simulink model "Powertrain_Comparison"  (R2024b)
settings: Solver=FixedStepDiscrete  StartTime=0.0  StopTime=3600  FixedStep=1  RelTol=1e-3
InitFcn:
  | try; sc=find_system(bdroot,'LookUnderMasks','all','FollowLinks','on','BlockType','Scope'); for k=1:numel(sc); c=get_param(sc{k},'ScopeConfiguration'); try; c.AxesScaling='Auto'; catch; end; try; nd=prod(c.LayoutDimensions); catch; nd=1; end; for d=1:nd; try; c.ActiveDisplay=d; catch; end; try; c.ShowLegend=true; catch; end; end; end; catch; end
(part 2 of 4)

== system Powertrain_Comparison/Electric powertrain/Battery DC converter ==
  note: Battery DC converter
  note: BIDIRECTIONAL DC CONVERTER | DC request to battery current
      | Reuses battery Voc and R. I = 2P / (Voc + sqrt(Voc^2 - 4RP)); avoids a terminal-voltage algebraic loop.
      | Bidirectional conversion and regenerative operation are route-model additions; conversion efficiency is assumed.
  note: INPUT SIGNALS
  note: PARAMETERS AND SIGNAL SELECTION
  note: CALCULATIONS AND CONTROL
  note: OUTPUTS AND MONITORING
  dispatch : Inport  PortDimensions=4
  fuel_cell_bus : Inport  Port=2  PortDimensions=3
  battery_state : Inport  Port=3  PortDimensions=12
  limits : Inport  Port=4  PortDimensions=2
  parameters : Inport  Port=5  PortDimensions=52
  Battery terminal power request W : Fcn  Expr=1000*((u(1)>=0)*u(1)/(((u(2))+(0.000001)+abs((u(2))-(0.000001)))/2)+(u(1)<0)*u(1)*u(2))
  Bus power within available current limits kW : Fcn  Expr=((((u(1))+(-u(3))+abs((u(1))-(-u(3))))/2)+(u(2))-abs((((u(1))+(-u(3))+abs((u(1))-(-u(3))))/2)-(u(2))))/2
  Ideal battery boost duty ratio : Fcn  Expr=((((1-u(1)/(((u(2))+(0.000001)+abs((u(2))-(0.000001)))/2))+(0)+abs((1-u(1)/(((u(2))+(0.000001)+abs((u(2))-(0.000001)))/2))-(0)))/2)+(0.95)-abs((((1-u(1)/(((u(2))+(0.000001)+abs((u(2))-(0.000001)))/2))+(0)+abs((1-u(1)/(((u(2))+(0.000001)+abs((u(2))-(0.000001)))/2))-(0)))/2)-(0.95)))/2
  Required battery bus power kW : Fcn  Expr=u(1)-u(2)
  Stable power-to-current request A : Fcn  Expr=2*u(1)/(((u(2)+sqrt(((u(2)^2-4*u(3)*u(1))+abs(u(2)^2-4*u(3)*u(1)))/2))+(0.000001)+abs((u(2)+sqrt(((u(2)^2-4*u(3)*u(1))+abs(u(2)^2-4*u(3)*u(1)))/2))-(0.000001)))/2)
  charge : Fcn  Expr=u(2)
  combine Converter request : Mux  Inputs=3
  combine Current command : Mux  Inputs=1
  dis : Fcn  Expr=u(1)
  eta_bconv : Fcn  Expr=u(27)
  fc : Fcn  Expr=u(1)
  inputs current_request : Mux  Inputs=3
  inputs duty : Mux  Inputs=2
  inputs limited : Mux  Inputs=3
  inputs request : Mux  Inputs=2
  inputs terminal : Mux  Inputs=2
  load : Fcn  Expr=u(4)
  r : Fcn  Expr=u(4)
  vbus : Fcn  Expr=u(25)
  voc : Fcn  Expr=u(3)
  Current command : Outport  PortDimensions=1
  Converter request : Outport  Port=2  PortDimensions=3
  wires:
  [r] -> inputs current_request/3
  [limits] -> charge/1
  [dispatch] -> load/1
  [fuel_cell_bus] -> fc/1
  [limited] -> combine Converter request/2
  [request] -> combine Converter request/1
  [parameters] -> eta_bconv/1
  [eta_bconv] -> inputs terminal/2
  [duty] -> combine Converter request/3
  [load] -> inputs request/1
  [request] -> inputs limited/1
  [limited] -> inputs terminal/1
  Bus power within available current limits kW/1 -> [limited]
  [voc] -> inputs duty/1
  limits/1 -> [limits]
  [vbus] -> inputs duty/2
  parameters/1 -> [parameters]
  dispatch/1 -> [dispatch]
  [fc] -> inputs request/2
  [terminal] -> inputs current_request/1
  [parameters] -> vbus/1
  [limits] -> dis/1
  battery_state/1 -> [battery_state]
  Battery terminal power request W/1 -> [terminal]
  [voc] -> inputs current_request/2
  inputs request/1 -> Required battery bus power kW/1
  r/1 -> [r]
  [current_request] -> combine Current command/1
  [battery_state] -> voc/1
  [dis] -> inputs limited/2
  [charge] -> inputs limited/3
  inputs terminal/1 -> Battery terminal power request W/1
  [battery_state] -> r/1
  fuel_cell_bus/1 -> [fuel_cell_bus]
  charge/1 -> [charge]
  combine Converter request/1 -> Converter request/1
  eta_bconv/1 -> [eta_bconv]
  load/1 -> [load]
  fc/1 -> [fc]
  Required battery bus power kW/1 -> [request]
  dis/1 -> [dis]
  vbus/1 -> [vbus]
  inputs current_request/1 -> Stable power-to-current request A/1
  combine Current command/1 -> Current command/1
  inputs limited/1 -> Bus power within available current limits kW/1
  inputs duty/1 -> Ideal battery boost duty ratio/1
  voc/1 -> [voc]
  Stable power-to-current request A/1 -> [current_request]
  Ideal battery boost duty ratio/1 -> [duty]

== system Powertrain_Comparison/Electric powertrain/Battery power limits ==
  note: Battery power limits
  note: BATTERY POWER LIMITS | state-dependent safe power at the DC bus
      | Pdis = (Voc - R Idis) Idis. Pcharge = (Voc + R Ich) Ich. The converter applies its directional efficiency.
  note: INPUT SIGNALS
  note: PARAMETERS AND SIGNAL SELECTION
  note: CALCULATIONS AND CONTROL
  note: OUTPUTS AND MONITORING
  demand : Inport  PortDimensions=12
  parameters : Inport  Port=2  PortDimensions=52
  Available bus charge sink kW : Fcn  Expr=(((u(1)+u(2)*u(3))*u(3)/(1000*(((u(4))+(0.000001)+abs((u(4))-(0.000001)))/2)))+abs((u(1)+u(2)*u(3))*u(3)/(1000*(((u(4))+(0.000001)+abs((u(4))-(0.000001)))/2))))/2
  Available bus discharge kW : Fcn  Expr=(((u(1)-u(2)*u(3))*u(3)*u(4)/1000)+abs((u(1)-u(2)*u(3))*u(3)*u(4)/1000))/2
  Current before maximum-power point A : Fcn  Expr=((u(1))+(u(2)/(2*(((u(3))+(0.000001)+abs((u(3))-(0.000001)))/2)))-abs((u(1))-(u(2)/(2*(((u(3))+(0.000001)+abs((u(3))-(0.000001)))/2)))))/2
  combine Power limits : Mux  Inputs=2
  eta_bconv : Fcn  Expr=u(27)
  ich : Fcn  Expr=u(6)
  idis : Fcn  Expr=u(5)
  inputs ch_bus : Mux
  inputs dis_bus : Mux
  inputs idis_safe : Mux  Inputs=3
  r : Fcn  Expr=u(4)
  voc : Fcn  Expr=u(3)
  Power limits : Outport  PortDimensions=2
  wires:
  [idis] -> inputs idis_safe/1
  [demand] -> voc/1
  [voc] -> inputs ch_bus/1
  inputs ch_bus/1 -> Available bus charge sink kW/1
  [voc] -> inputs dis_bus/1
  [ich] -> inputs ch_bus/3
  [ch_bus] -> combine Power limits/2
  idis/1 -> [idis]
  [r] -> inputs dis_bus/2
  [dis_bus] -> combine Power limits/1
  inputs dis_bus/1 -> Available bus discharge kW/1
  [demand] -> idis/1
  [parameters] -> eta_bconv/1
  [idis_safe] -> inputs dis_bus/3
  [demand] -> r/1
  demand/1 -> [demand]
  inputs idis_safe/1 -> Current before maximum-power point A/1
  [eta_bconv] -> inputs dis_bus/4
  [r] -> inputs ch_bus/2
  r/1 -> [r]
  [voc] -> inputs idis_safe/2
  [eta_bconv] -> inputs ch_bus/4
  eta_bconv/1 -> [eta_bconv]
  parameters/1 -> [parameters]
  [demand] -> ich/1
  [r] -> inputs idis_safe/3
  voc/1 -> [voc]
  combine Power limits/1 -> Power limits/1
  ich/1 -> [ich]
  Available bus charge sink kW/1 -> [ch_bus]
  Current before maximum-power point A/1 -> [idis_safe]
  Available bus discharge kW/1 -> [dis_bus]

== system Powertrain_Comparison/Electric powertrain/Battery storage ==
  note: Battery storage
  note: BATTERY STORAGE | reused battery-management model
      | Open Battery management to edit its pack mask. Current positive = discharge, negative = charge.
      | State output contains delayed SOC/temperature and state-derived limits; actual output contains delivered current, voltage and
      | power.
  note: INPUT SIGNALS
  note: CALCULATIONS AND CONTROL
  note: OUTPUTS AND MONITORING
  current_request : Inport  PortDimensions=1
  ambient : Inport  Port=2  PortDimensions=1
  Battery management : Subsystem  Description=Copied and adapted native battery energy-management subsystem. 96s41p; nominal59.51232kWh. SOC, OCV, current restrictions, I2R losses, thermal state, terminal energy and exact OCV-based stored energy. All data remain illustrative. No external file dependencies.  mask(Battery management parameters){initial_soc_pct=90, initial_temp_C=25, ns=96, np=41, cell_capacity_Ah=4.2, cell_nominal_V=3.6, cell_resistance_ohm=0.016, cell_voltage_limits_V=[2.5 4.2], current_ratings_C=[2 2], soc_levels_pct=[15 20 80 95], charge_temp_limits_C=[0 10 35 45], discharge_temp_limits_C=[-20 0 45 55], mass_kg=341.6666666667, cp_J_kgK=900, conductance_W_K=35, coulombic_efficiencies=[1 1], ocv_soc_pct=[0 5 10 20 30 40 50 60 70 80 90 95 100], ocv_cell_V=[2.5 3.1 3.3 3.45 3.53 3.6 3.67 3.73 3.8 3.9 4.04 4.12 4.2]}
      mask prompts: initial_soc_pct "Initial state of charge (%)"; initial_temp_C "Initial battery temperature (degC)"; ns "Series-connected cell groups, Ns"; np "Parallel cells per group, Np"; cell_capacity_Ah "Capacity of ONE cell (Ah)"; cell_nominal_V "Nominal voltage of ONE cell (V)"; cell_resistance_ohm "Resistance of ONE cell (ohm)"; cell_voltage_limits_V "Cell voltage limits [minimum maximum] (V)"; current_ratings_C "Current ratings [charge discharge] (C-rate)"; soc_levels_pct "SOC levels [minimum reserve taper maximum] (%)"; charge_temp_limits_C "Charge temperatures [stop-low full-low full-high stop-high] (degC)"; discharge_temp_limits_C "Discharge temperatures [stop-low full-low full-high stop-high] (degC)"; mass_kg "Effective pack thermal mass (kg)"; cp_J_kgK "Effective specific heat (J/(kg.K))"; conductance_W_K "Heat transfer to ambient (W/K)"; coulombic_efficiencies "Coulombic efficiencies [charge discharge] (0 to 1)"; ocv_soc_pct "OCV lookup: SOC breakpoints (%)"; ocv_cell_V "OCV lookup: matching single-cell voltages (V)"
      mask help: Reused battery-management model. Positive current discharges; negative current charges. Defaults use a96s41p,59.51232kWh nominal pack. OCV, resistance, thermal data and operating limits are illustrative. Keep13 OCV points. Fixed sample time1s. Stop simulation before changing data.
      mask init:
      | % Embedded parameter definitions. This code is stored in the SLX, not an external file.
      | assert(isscalar(ns) && isfinite(ns) && ns>=1 && ns==fix(ns), 'Series groups must be a positive integer.');
      | assert(isscalar(np) && isfinite(np) && np>=1 && np==fix(np), 'Parallel cells must be a positive integer.');
      | assert(isscalar(cell_capacity_Ah) && isfinite(cell_capacity_Ah) && cell_capacity_Ah>0, 'Cell capacity must be positive.');
      | assert(isscalar(cell_nominal_V) && isfinite(cell_nominal_V) && cell_nominal_V>0, 'Nominal cell voltage must be positive.');
      | assert(isscalar(cell_resistance_ohm) && isfinite(cell_resistance_ohm) && cell_resistance_ohm>0, 'Cell resistance must be greater than zero.');
      | assert(numel(cell_voltage_limits_V)==2 && all(isfinite(cell_voltage_limits_V)) && cell_voltage_limits_V(1)>0 && cell_voltage_limits_V(2)>cell_voltage_limits_V(1), 'Enter increasing positive cell voltage limits [min max].');
      | assert(cell_nominal_V>=cell_voltage_limits_V(1) && cell_nominal_V<=cell_voltage_limits_V(2), 'Nominal voltage must lie within the cell voltage limits.');
      | assert(numel(current_ratings_C)==2 && all(isfinite(current_ratings_C)) && all(current_ratings_C>=0), 'Enter two nonnegative C-rates [charge discharge].');
      | assert(numel(soc_levels_pct)==4 && all(isfinite(soc_levels_pct)) && all(diff(soc_levels_pct)>0) && soc_levels_pct(1)>=0 && soc_levels_pct(4)<=100, 'SOC levels must increase: minimum < reserve < taper < maximum, within 0 to 100.');
      | assert(isscalar(initial_soc_pct) && isfinite(initial_soc_pct) && initial_soc_pct>=soc_levels_pct(1) && initial_soc_pct<=soc_levels_pct(4), 'Initial SOC must lie inside the operating SOC window.');
      | assert(isscalar(initial_temp_C) && isfinite(initial_temp_C), 'Initial temperature must be a finite scalar.');
      | assert(numel(charge_temp_limits_C)==4 && all(isfinite(charge_temp_limits_C)) && all(diff(charge_temp_limits_C)>0), 'Enter four increasing charge-temperature limits.');
      | assert(numel(discharge_temp_limits_C)==4 && all(isfinite(discharge_temp_limits_C)) && all(diff(discharge_temp_limits_C)>0), 'Enter four increasing discharge-temperature limits.');
      | assert(isscalar(mass_kg) && isfinite(mass_kg) && mass_kg>0 && isscalar(cp_J_kgK) && isfinite(cp_J_kgK) && cp_J_kgK>0, 'Mass and specific heat must be positive.');
      | assert(isscalar(conductance_W_K) && isfinite(conductance_W_K) && conductance_W_K>=0, 'Ambient conductance must not be negative.');
      | assert(numel(coulombic_efficiencies)==2 && all(isfinite(coulombic_efficiencies)) && all(coulombic_efficiencies>0) && all(coulombic_efficiencies<=1), 'Coulombic efficiencies must be in (0,1].');
      | assert(isvector(ocv_soc_pct) && isvector(ocv_cell_V) && numel(ocv_soc_pct)>=2 && numel(ocv_soc_pct)==numel(ocv_cell_V), 'OCV arrays must be equal-length vectors.');
      | assert(all(isfinite(ocv_soc_pct)) && all(isfinite(ocv_cell_V)) && all(diff(ocv_soc_pct)>0) && ocv_soc_pct(1)==0 && ocv_soc_pct(end)==100, 'OCV SOC breakpoints must increase from 0 to 100.');
      | assert(all(diff(ocv_cell_V)>=0) && all(ocv_cell_V>=cell_voltage_limits_V(1)) && all(ocv_cell_V<=cell_voltage_limits_V(2)), 'OCV voltages must be nondecreasing and within the cell voltage limits.');
      | initial_soc=initial_soc_pct/100;
      | soc_min=soc_levels_pct(1)/100; soc_reserve=soc_levels_pct(2)/100;
      | soc_taper=soc_levels_pct(3)/100; soc_max=soc_levels_pct(4)/100;
      | cell_min_V=cell_voltage_limits_V(1); cell_max_V=cell_voltage_limits_V(2);
      | charge_rate_C=current_ratings_C(1); discharge_rate_C=current_ratings_C(2);
      | charge_T1_C=charge_temp_limits_C(1); charge_T2_C=charge_temp_limits_C(2);
      | charge_T3_C=charge_temp_limits_C(3); charge_T4_C=charge_temp_limits_C(4);
      | discharge_T1_C=discharge_temp_limits_C(1); discharge_T2_C=discharge_temp_limits_C(2);
      | discharge_T3_C=discharge_temp_limits_C(3); discharge_T4_C=discharge_temp_limits_C(4);
      | eta_charge=coulombic_efficiencies(1); eta_discharge=coulombic_efficiencies(2);
      | ocv_soc=ocv_soc_pct/100;
      | dt_s=1;
      | 
      | % Added exact OCV-integral energy accounting for the comparison.
      | assert(numel(ocv_soc)==13, 'This version requires13 OCV breakpoints and13 voltages.');
      | ocv_soc = reshape(ocv_soc,1,[]);
      | ocv_cell_V = reshape(ocv_cell_V,1,[]);
      | energy_s = [ocv_soc(ocv_soc<initial_soc) initial_soc];
      | energy_v = interp1(ocv_soc,ocv_cell_V,energy_s,'linear');
      | initial_stored_energy_kWh = ns*np*cell_capacity_Ah*trapz(energy_s,energy_v)/1000;
      mask Display: disp('BATTERY MANAGEMENT\n\nSOC and temperature\nVoltage and current limits\nLosses and energy\n\nDouble-click: parameters')
  combine Battery actual : Mux  Inputs=7
  combine Battery state : Mux  Inputs=12
  Battery state : Outport  PortDimensions=12
  Battery actual : Outport  Port=2  PortDimensions=7
  wires:
  current_request/1 -> [current_request]
  ambient/1 -> [ambient]
  [b8] -> combine Battery actual/2
  [b10] -> combine Battery actual/4
  [b6] -> combine Battery state/6
  [ambient] -> Battery management/2(AMBIENT_C)
  [b12] -> combine Battery actual/6
  [current_request] -> Battery management/1(CURRENT_A)
  [b11] -> combine Battery actual/5
  [b9] -> combine Battery actual/3
  [b1] -> combine Battery state/1
  [b7] -> combine Battery actual/1
  [b19] -> combine Battery actual/7
  [b2] -> combine Battery state/2
  [b3] -> combine Battery state/3
  [b4] -> combine Battery state/4
  [b5] -> combine Battery state/5
  [b13] -> combine Battery state/7
  [b14] -> combine Battery state/8
  [b15] -> combine Battery state/9
  [b16] -> combine Battery state/10
  [b17] -> combine Battery state/11
  [b18] -> combine Battery state/12
  Battery management/17(Stored_energy_kWh) -> [b17]
  Battery management/1(SOC_fraction) -> [b1]
  Battery management/18(Initial_stored_energy_kWh) -> [b18]
  Battery management/2(Battery_temperature_C) -> [b2]
  Battery management/19(Ohmic_loss_energy_kWh) -> [b19]
  Battery management/3(Open_circuit_voltage_V) -> [b3]
  Battery management/4(Equivalent_resistance_ohm) -> [b4]
  Battery management/5(Discharge_limit_A) -> [b5]
  Battery management/6(Charge_limit_A) -> [b6]
  Battery management/7(Terminal_voltage_V) -> [b7]
  Battery management/8(Actual_current_A) -> [b8]
  Battery management/9(Terminal_power_W) -> [b9]
  Battery management/10(Discharged_energy_kWh) -> [b10]
  Battery management/11(Charged_energy_kWh) -> [b11]
  Battery management/12(Ohmic_heat_W) -> [b12]
  Battery management/13(Initial_SOC_fraction) -> [b13]
  Battery management/14(Nominal_energy_kWh) -> [b14]
  Battery management/15(Capacity_Ah) -> [b15]
  Battery management/16(Stored_energy_depletion_kWh) -> [b16]
  combine Battery actual/1 -> Battery actual/1
  combine Battery state/1 -> Battery state/1

== system Powertrain_Comparison/Electric powertrain/DC boost converter ==
  note: DC boost converter
  note: DC BOOST CONVERTER | fuel-cell module to regulated DC link
      | Reuses boost steady-state Vout = Vin / (1-D). Dynamic switching and fixed resistive bench load are replaced by bus demand.
  note: INPUT SIGNALS
  note: PARAMETERS AND SIGNAL SELECTION
  note: CALCULATIONS AND CONTROL
  note: OUTPUTS AND MONITORING
  demand : Inport  PortDimensions=3
  parameters : Inport  Port=2  PortDimensions=52
  Boost converter loss kW : Fcn  Expr=u(1)-u(2)
  Fuel cell delivered DC bus kW : Fcn  Expr=u(1)*u(2)
  Ideal boost duty ratio : Fcn  Expr=((((1-u(1)/(((u(2))+(0.000001)+abs((u(2))-(0.000001)))/2))+(0)+abs((1-u(1)/(((u(2))+(0.000001)+abs((u(2))-(0.000001)))/2))-(0)))/2)+(0.95)-abs((((1-u(1)/(((u(2))+(0.000001)+abs((u(2))-(0.000001)))/2))+(0)+abs((1-u(1)/(((u(2))+(0.000001)+abs((u(2))-(0.000001)))/2))-(0)))/2)-(0.95)))/2
  combine Converter signals : Mux  Inputs=3
  eta_fcconv : Fcn  Expr=u(30)
  fc_voltage : Fcn  Expr=u(52)
  inputs bus : Mux  Inputs=2
  inputs duty : Mux  Inputs=2
  inputs loss : Mux  Inputs=2
  module : Fcn  Expr=u(1)
  vbus : Fcn  Expr=u(25)
  Converter signals : Outport  PortDimensions=3
  wires:
  [module] -> inputs bus/1
  [parameters] -> eta_fcconv/1
  [parameters] -> vbus/1
  [duty] -> combine Converter signals/3
  [bus] -> combine Converter signals/1
  Ideal boost duty ratio/1 -> [duty]
  [demand] -> module/1
  eta_fcconv/1 -> [eta_fcconv]
  [loss] -> combine Converter signals/2
  parameters/1 -> [parameters]
  [eta_fcconv] -> inputs bus/2
  [module] -> inputs loss/1
  [bus] -> inputs loss/2
  combine Converter signals/1 -> Converter signals/1
  [fc_voltage] -> inputs duty/1
  [vbus] -> inputs duty/2
  inputs duty/1 -> Ideal boost duty ratio/1
  demand/1 -> [demand]
  [parameters] -> fc_voltage/1
  Boost converter loss kW/1 -> [loss]
  module/1 -> [module]
  vbus/1 -> [vbus]
  inputs bus/1 -> Fuel cell delivered DC bus kW/1
  inputs loss/1 -> Boost converter loss kW/1
  fc_voltage/1 -> [fc_voltage]
  Fuel cell delivered DC bus kW/1 -> [bus]

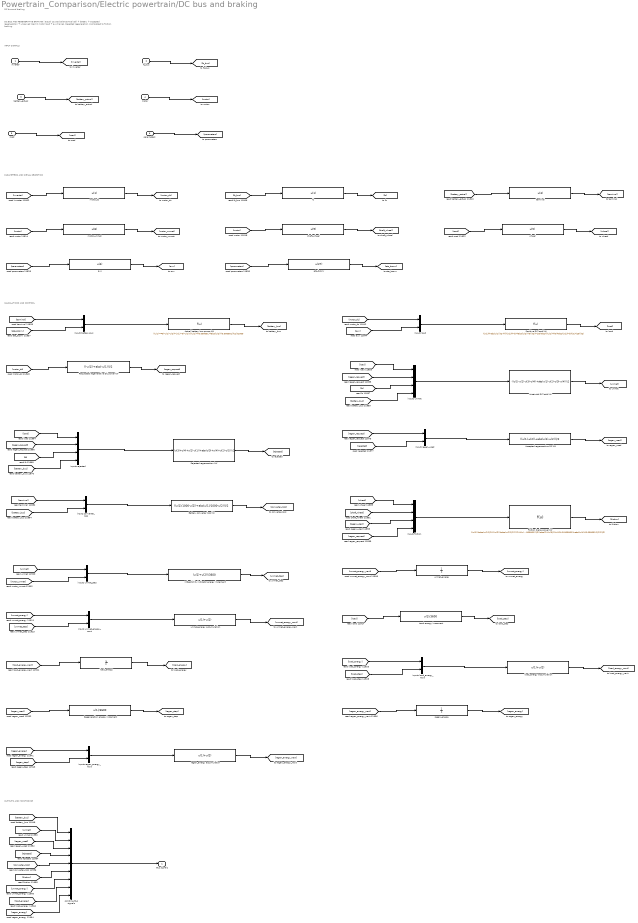
== system Powertrain_Comparison/Electric powertrain/DC bus and braking ==
  note: DC bus and braking
  note: DC BUS AND REGENERATIVE BRAKING | actual source balance
      | Fuel cell + battery + accepted regeneration + unserved load = motor load + auxiliaries. Rejected regeneration is allocated to
      | friction braking.
  note: INPUT SIGNALS
  note: PARAMETERS AND SIGNAL SELECTION
  note: CALCULATIONS AND CONTROL
  note: OUTPUTS AND MONITORING
  inverter : Inport  PortDimensions=2
  fc_bus : Inport  Port=2  PortDimensions=3
  battery_actual : Inport  Port=3  PortDimensions=7
  motor : Inport  Port=4  PortDimensions=9
  road : Inport  Port=5  PortDimensions=9
  parameters : Inport  Port=6  PortDimensions=52
  Accepted regenerative DC kW : Fcn  Expr=((u(1)-u(2))+abs(u(1)-u(2)))/2
  Actual battery bus power kW : Fcn  Expr=((u(1)>=0)*u(1)*u(2)+(u(1)<0)*u(1)/(((u(2))+(0.000001)+abs((u(2))-(0.000001)))/2))/1000
  Battery converter loss kW : Fcn  Expr=((u(1)/1000-u(2))+abs(u(1)/1000-u(2)))/2
  Friction brake power kW : Fcn  Expr=((-u(1))+abs(-u(1)))/2-(((-u(2))+abs(-u(2)))/2)*(((1)+(u(3)/(((u(4))+(0.000001)+abs((u(4))-(0.000001)))/2))-abs((1)-(u(3)/(((u(4))+(0.000001)+abs((u(4))-(0.000001)))/2))))/2)
  Infeasibility indicator energy increment : Fcn  Expr=(u(1)+u(2))/3600
  Load energy increment : Fcn  Expr=u(1)/3600
  Positive DC load kW : Fcn  Expr=((u(1))+abs(u(1)))/2+(((((u(2))+(0)+abs((u(2))-(0)))/2)+(20)-abs((((u(2))+(0)+abs((u(2))-(0)))/2)-(20)))/2)
  Regeneration energy increment : Fcn  Expr=u(1)/3600
  Rejected regeneration kW : Fcn  Expr=((u(3)+u(4)+u(2)-u(1))+abs(u(3)+u(4)+u(2)-u(1)))/2
  Requested regenerative DC power kW : Fcn  Expr=((-u(1))+abs(-u(1)))/2
  Unserved DC load kW : Fcn  Expr=((u(1)-u(2)-u(3)-u(4))+abs(u(1)-u(2)-u(3)-u(4)))/2
  aux : Fcn  Expr=u(4)
  combine Bus signals : Mux  Inputs=9
  eta_bconv : Fcn  Expr=u(27)
  fc : Fcn  Expr=u(1)
  inputs battery_bus : Mux  Inputs=2
  inputs converter_loss : Mux  Inputs=2
  inputs friction : Mux
  inputs load : Mux  Inputs=2
  inputs load_energy_next : Mux  Inputs=2
  inputs regen_energy_next : Mux  Inputs=2
  inputs regen_used : Mux  Inputs=2
  inputs rejected : Mux
  inputs unmet : Mux
  inputs unmet_energy_next : Mux  Inputs=2
  inputs unmet_step : Mux  Inputs=2
  load_energy : UnitDelay
  load_energy accumulation : Fcn  Expr=u(1)+u(2)
  motor_dc : Fcn  Expr=u(1)
  motor_unmet : Fcn  Expr=u(8)
  regen_energy : UnitDelay
  regen_energy accumulation : Fcn  Expr=u(1)+u(2)
  shaft_wheel : Fcn  Expr=u(9)
  terminal : Fcn  Expr=u(3)
  unmet_energy : UnitDelay
  unmet_energy accumulation : Fcn  Expr=u(1)+u(2)
  wheel : Fcn  Expr=u(5)
  Bus signals : Outport  PortDimensions=9
  wires:
  [motor_dc] -> inputs load/1
  [rejected] -> inputs regen_used/2
  [converter_loss] -> combine Bus signals/5
  [regen_used] -> Regeneration energy increment/1
  [battery_bus] -> inputs converter_loss/2
  [motor] -> motor_unmet/1
  motor_unmet/1 -> [motor_unmet]
  [regen_request] -> inputs rejected/2
  [load] -> Load energy increment/1
  [unmet_energy] -> combine Bus signals/7
  [terminal] -> inputs converter_loss/1
  [regen_energy] -> inputs regen_energy_next/1
  [friction] -> combine Bus signals/6
  [motor_dc] -> Requested regenerative DC power kW/1
  [eta_bconv] -> inputs battery_bus/2
  [rejected] -> combine Bus signals/4
  [motor] -> shaft_wheel/1
  [battery_bus] -> combine Bus signals/1
  [regen_used] -> combine Bus signals/3
  [regen_energy_next] -> regen_energy/1
  [load] -> inputs unmet/1
  [unmet] -> combine Bus signals/2
  [regen_request] -> inputs friction/4
  [unmet_step] -> inputs unmet_energy_next/2
  [battery_actual] -> terminal/1
  [load_energy] -> combine Bus signals/8
  [unmet] -> inputs unmet_step/1
  [inverter] -> motor_dc/1
  [regen_energy] -> combine Bus signals/9
  [aux] -> inputs load/2
  [unmet_energy_next] -> unmet_energy/1
  [regen_request] -> inputs regen_used/1
  [load_energy] -> inputs load_energy_next/1
  [battery_bus] -> inputs rejected/4
  [regen_used] -> inputs friction/3
  [load_step] -> inputs load_energy_next/2
  [terminal] -> inputs battery_bus/1
  [parameters] -> eta_bconv/1
  [fc_bus] -> fc/1
  parameters/1 -> [parameters]
  [road] -> wheel/1
  [fc] -> inputs unmet/3
  [motor_unmet] -> inputs unmet_step/2
  [wheel] -> inputs friction/1
  [load_energy_next] -> load_energy/1
  [battery_bus] -> inputs unmet/4
  [regen_step] -> inputs regen_energy_next/2
  [load] -> inputs rejected/1
  [unmet_energy] -> inputs unmet_energy_next/1
  [regen_request] -> inputs unmet/2
  inverter/1 -> [inverter]
  motor/1 -> [motor]
  battery_actual/1 -> [battery_actual]
  road/1 -> [road]
  [fc] -> inputs rejected/3
  [shaft_wheel] -> inputs friction/2
  [parameters] -> aux/1
  fc_bus/1 -> [fc_bus]
  combine Bus signals/1 -> Bus signals/1
  inputs load_energy_next/1 -> load_energy accumulation/1
  fc/1 -> [fc]
  motor_dc/1 -> [motor_dc]
  inputs unmet_step/1 -> Infeasibility indicator energy increment/1
  inputs regen_energy_next/1 -> regen_energy accumulation/1
  inputs unmet/1 -> Unserved DC load kW/1
  shaft_wheel/1 -> [shaft_wheel]
  wheel/1 -> [wheel]
  load_energy/1 -> [load_energy]
  terminal/1 -> [terminal]
  inputs unmet_energy_next/1 -> unmet_energy accumulation/1
  eta_bconv/1 -> [eta_bconv]
  regen_energy/1 -> [regen_energy]
  inputs regen_used/1 -> Accepted regenerative DC kW/1
  unmet_energy/1 -> [unmet_energy]
  inputs battery_bus/1 -> Actual battery bus power kW/1
  Requested regenerative DC power kW/1 -> [regen_request]
  aux/1 -> [aux]
  inputs friction/1 -> Friction brake power kW/1
  inputs load/1 -> Positive DC load kW/1
  inputs converter_loss/1 -> Battery converter loss kW/1
  Load energy increment/1 -> [load_step]
  Regeneration energy increment/1 -> [regen_step]
  inputs rejected/1 -> Rejected regeneration kW/1
  load_energy accumulation/1 -> [load_energy_next]
  Infeasibility indicator energy increment/1 -> [unmet_step]
  regen_energy accumulation/1 -> [regen_energy_next]
  Unserved DC load kW/1 -> [unmet]
  unmet_energy accumulation/1 -> [unmet_energy_next]
  Accepted regenerative DC kW/1 -> [regen_used]
  Actual battery bus power kW/1 -> [battery_bus]
  Friction brake power kW/1 -> [friction]
  Positive DC load kW/1 -> [load]
  Battery converter loss kW/1 -> [converter_loss]
  Rejected regeneration kW/1 -> [rejected]

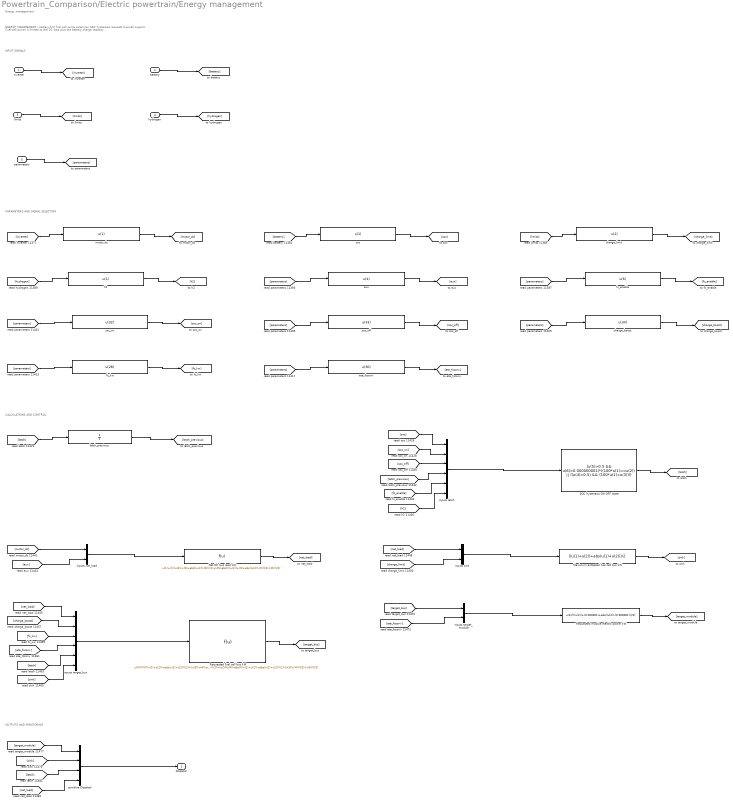
== system Powertrain_Comparison/Electric powertrain/Energy management ==
  note: Energy management
  note: ENERGY MANAGEMENT | battery-first fuel-cell range extension
      | SOC hysteresis requests fuel-cell support. Fuel-cell power is limited to the DC load plus the battery charge capacity.
  note: INPUT SIGNALS
  note: PARAMETERS AND SIGNAL SELECTION
  note: CALCULATIONS AND CONTROL
  note: OUTPUTS AND MONITORING
  inverter : Inport  PortDimensions=2
  battery : Inport  Port=2  PortDimensions=12
  limits : Inport  Port=3  PortDimensions=2
  hydrogen : Inport  Port=4  PortDimensions=3
  parameters : Inport  Port=5  PortDimensions=52
  Maximum accepted fuel cell bus kW : Fcn  Expr=((u(1)+u(2))+abs(u(1)+u(2)))/2
  Net DC bus load kW : Fcn  Expr=u(1)+(((((u(2))+(0)+abs((u(2))-(0)))/2)+(20)-abs((((u(2))+(0)+abs((u(2))-(0)))/2)-(20)))/2)
  Requested fuel cell bus kW : Fcn  Expr=u(5)*(((((((u(1)+u(2))+abs(u(1)+u(2)))/2)+(u(3)*u(4))-abs((((u(1)+u(2))+abs(u(1)+u(2)))/2)-(u(3)*u(4))))/2)+(u(6))-abs((((((u(1)+u(2))+abs(u(1)+u(2)))/2)+(u(3)*u(4))-abs((((u(1)+u(2))+abs(u(1)+u(2)))/2)-(u(3)*u(4))))/2)-(u(6))))/2)
  Requested module electric power kW : Fcn  Expr=u(1)/(((u(2))+(0.000001)+abs((u(2))-(0.000001)))/2)
  SOC hysteresis ON OFF state : Fcn  Expr=(u(5)>0.5 && u(6)>0.000000001)*((100*u(1)<=u(2)) || ((u(4)>0.5) && (100*u(1)<u(3))))
  aux : Fcn  Expr=u(4)
  charge_boost : Fcn  Expr=u(34)
  charge_limit : Fcn  Expr=u(2)
  combine Dispatch : Mux
  eta_fcconv : Fcn  Expr=u(30)
  fc_enable : Fcn  Expr=u(6)
  fc_kw : Fcn  Expr=u(28)
  h2 : Fcn  Expr=u(1)
  inputs latch : Mux  Inputs=6
  inputs net_load : Mux  Inputs=2
  inputs sink : Mux  Inputs=2
  inputs target_bus : Mux  Inputs=6
  inputs target_module : Mux  Inputs=2
  latch_previous : UnitDelay
  motor_dc : Fcn  Expr=u(1)
  soc : Fcn  Expr=u(1)
  soc_off : Fcn  Expr=u(33)
  soc_on : Fcn  Expr=u(32)
  Dispatch : Outport  PortDimensions=4
  wires:
  inputs sink/1 -> Maximum accepted fuel cell bus kW/1
  limits/1 -> [limits]
  inputs target_bus/1 -> Requested fuel cell bus kW/1
  parameters/1 -> [parameters]
  [fc_enable] -> inputs latch/5
  [parameters] -> soc_on/1
  [aux] -> inputs net_load/2
  [motor_dc] -> inputs net_load/1
  [target_bus] -> inputs target_module/1
  soc_off/1 -> [soc_off]
  [eta_fcconv] -> inputs target_bus/4
  [parameters] -> aux/1
  [eta_fcconv] -> inputs target_module/2
  [parameters] -> fc_enable/1
  [soc_on] -> inputs latch/2
  [limits] -> charge_limit/1
  [inverter] -> motor_dc/1
  [parameters] -> eta_fcconv/1
  [h2] -> inputs latch/6
  [parameters] -> charge_boost/1
  [parameters] -> fc_kw/1
  [hydrogen] -> h2/1
  [fc_kw] -> inputs target_bus/3
  [parameters] -> soc_off/1
  [latch] -> combine Dispatch/3
  [soc] -> inputs latch/1
  [latch_previous] -> inputs latch/4
  [soc_off] -> inputs latch/3
  [battery] -> soc/1
  [target_module] -> combine Dispatch/1
  [net_load] -> inputs sink/1
  [net_load] -> combine Dispatch/4
  [charge_limit] -> inputs sink/2
  battery/1 -> [battery]
  [latch] -> inputs target_bus/5
  [sink] -> combine Dispatch/2
  [charge_boost] -> inputs target_bus/2
  [net_load] -> inputs target_bus/1
  [latch] -> latch_previous/1
  [sink] -> inputs target_bus/6
  inputs net_load/1 -> Net DC bus load kW/1
  charge_limit/1 -> [charge_limit]
  inverter/1 -> [inverter]
  combine Dispatch/1 -> Dispatch/1
  hydrogen/1 -> [hydrogen]
  aux/1 -> [aux]
  inputs target_module/1 -> Requested module electric power kW/1
  soc_on/1 -> [soc_on]
  fc_enable/1 -> [fc_enable]
  eta_fcconv/1 -> [eta_fcconv]
  charge_boost/1 -> [charge_boost]
  h2/1 -> [h2]
  inputs latch/1 -> SOC hysteresis ON OFF state/1
  Requested module electric power kW/1 -> [target_module]
  motor_dc/1 -> [motor_dc]
  fc_kw/1 -> [fc_kw]
  soc/1 -> [soc]
  Requested fuel cell bus kW/1 -> [target_bus]
  latch_previous/1 -> [latch_previous]
  SOC hysteresis ON OFF state/1 -> [latch]
  Maximum accepted fuel cell bus kW/1 -> [sink]
  Net DC bus load kW/1 -> [net_load]

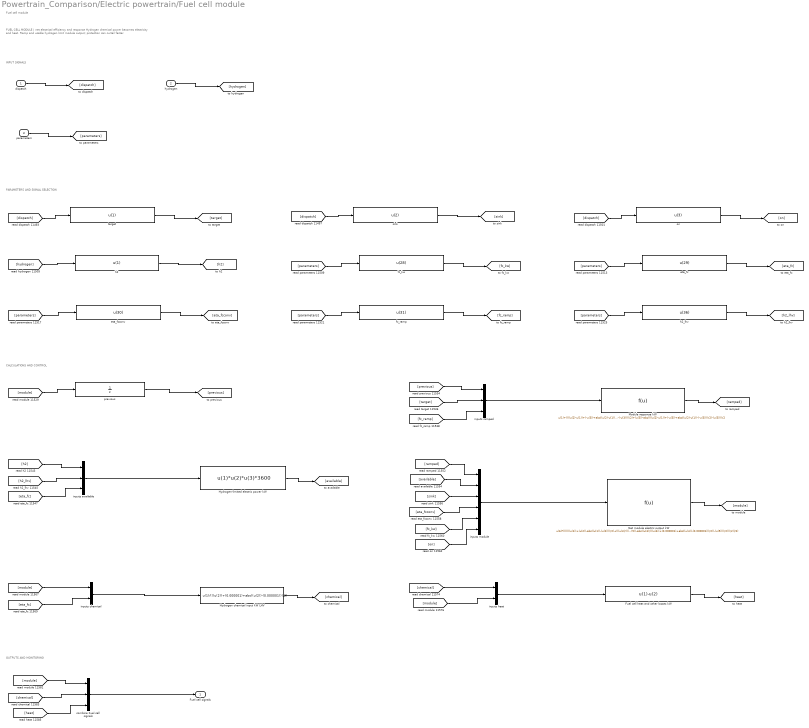
== system Powertrain_Comparison/Electric powertrain/Fuel cell module ==
  note: Fuel cell module
  note: FUEL CELL MODULE | net electrical efficiency and response
      | Hydrogen chemical power becomes electricity and heat. Ramp and usable hydrogen limit module output; protection can curtail
      | faster.
  note: INPUT SIGNALS
  note: PARAMETERS AND SIGNAL SELECTION
  note: CALCULATIONS AND CONTROL
  note: OUTPUTS AND MONITORING
  dispatch : Inport  PortDimensions=4
  hydrogen : Inport  Port=2  PortDimensions=3
  parameters : Inport  Port=3  PortDimensions=52
  Fuel cell heat and other losses kW : Fcn  Expr=u(1)-u(2)
  Hydrogen chemical input kW LHV : Fcn  Expr=u(1)/(((u(2))+(0.000001)+abs((u(2))-(0.000001)))/2)
  Hydrogen-limited electric power kW : Fcn  Expr=u(1)*u(2)*u(3)*3600
  Module response kW : Fcn  Expr=u(1)+((((u(2)-u(1))+(-u(3))+abs((u(2)-u(1))-(-u(3))))/2)+(u(3))-abs((((u(2)-u(1))+(-u(3))+abs((u(2)-u(1))-(-u(3))))/2)-(u(3))))/2
  Net module electric output kW : Fcn  Expr=u(6)*(((((((u(1))+(u(2))-abs((u(1))-(u(2))))/2)+(((u(3)/(((u(4))+(0.000001)+abs((u(4))-(0.000001)))/2))+(u(5))-abs((u(3)/(((u(4))+(0.000001)+abs((u(4))-(0.000001)))/2))-(u(5))))/2)-abs((((u(1))+(u(2))-abs((u(1))-(u(2))))/2)-(((u(3)/(((u(4))+(0.000001)+abs((u(4))-(0.000001)))/2))+(u(5))-abs((u(3)/(((u(4))+(0.000001)+abs((u(4))-(0.000001)))/2))-(u(5))))/2)))/2)+abs(((((u(1))+(u(2))-abs((u(1))-(u(2))))/2)+(((u(3)/(((u(4))+(0.000001)+abs((u(4))-(0.000001)))/2))+(u(5))-abs((u(3)/(((u(4))+(0.000001)+abs((u(4))-(0.000001)))/2))-(u(5))))/2)-abs((((u(1))+(u(2))-abs((u(1))-(u(2))))/2)-(((u(3)/(((u(4))+(0.000001)+abs((u(4))-(0.000001)))/2))+(u(5))-abs((u(3)/(((u(4))+(0.000001)+abs((u(4))-(0.000001)))/2))-(u(5))))/2)))/2))/2)
  combine Fuel cell signals : Mux  Inputs=3
  eta_fc : Fcn  Expr=u(29)
  eta_fcconv : Fcn  Expr=u(30)
  fc_kw : Fcn  Expr=u(28)
  fc_ramp : Fcn  Expr=u(31)
  h2 : Fcn  Expr=u(1)
  h2_lhv : Fcn  Expr=u(36)
  inputs available : Mux  Inputs=3
  inputs chemical : Mux  Inputs=2
  inputs heat : Mux  Inputs=2
  inputs module : Mux  Inputs=6
  inputs ramped : Mux  Inputs=3
  on : Fcn  Expr=u(3)
  previous : UnitDelay
  sink : Fcn  Expr=u(2)
  target : Fcn  Expr=u(1)
  Fuel cell signals : Outport  PortDimensions=3
  wires:
  [previous] -> inputs ramped/1
  [parameters] -> eta_fc/1
  [target] -> inputs ramped/2
  [parameters] -> fc_kw/1
  hydrogen/1 -> [hydrogen]
  [hydrogen] -> h2/1
  [fc_ramp] -> inputs ramped/3
  [parameters] -> fc_ramp/1
  [parameters] -> eta_fcconv/1
  [dispatch] -> on/1
  [module] -> combine Fuel cell signals/1
  [chemical] -> combine Fuel cell signals/2
  [heat] -> combine Fuel cell signals/3
  [h2] -> inputs available/1
  [h2_lhv] -> inputs available/2
  [eta_fc] -> inputs available/3
  [dispatch] -> sink/1
  [chemical] -> inputs heat/1
  [module] -> inputs heat/2
  [parameters] -> h2_lhv/1
  fc_ramp/1 -> [fc_ramp]
  parameters/1 -> [parameters]
  [ramped] -> inputs module/1
  [available] -> inputs module/2
  [sink] -> inputs module/3
  [eta_fcconv] -> inputs module/4
  [fc_kw] -> inputs module/5
  [on] -> inputs module/6
  [dispatch] -> target/1
  [module] -> inputs chemical/1
  [eta_fc] -> inputs chemical/2
  dispatch/1 -> [dispatch]
  [module] -> previous/1
  eta_fc/1 -> [eta_fc]
  fc_kw/1 -> [fc_kw]
  inputs ramped/1 -> Module response kW/1
  Fuel cell heat and other losses kW/1 -> [heat]
  h2/1 -> [h2]
  eta_fcconv/1 -> [eta_fcconv]
  inputs chemical/1 -> Hydrogen chemical input kW LHV/1
  sink/1 -> [sink]
  on/1 -> [on]
  inputs heat/1 -> Fuel cell heat and other losses kW/1
  combine Fuel cell signals/1 -> Fuel cell signals/1
  Module response kW/1 -> [ramped]
  inputs available/1 -> Hydrogen-limited electric power kW/1
  Hydrogen chemical input kW LHV/1 -> [chemical]
  h2_lhv/1 -> [h2_lhv]
  inputs module/1 -> Net module electric output kW/1
  previous/1 -> [previous]
  target/1 -> [target]
  Hydrogen-limited electric power kW/1 -> [available]
  Net module electric output kW/1 -> [module]

== system Powertrain_Comparison/Electric powertrain/Hydrogen storage ==
  note: Hydrogen storage
  note: HYDROGEN STORAGE | usable inventory
      | Hydrogen flow = module chemical input / LHV. This models usable mass and energy, not tank pressure or filling transients.
  note: INPUT SIGNALS
  note: PARAMETERS AND SIGNAL SELECTION
  note: CALCULATIONS AND CONTROL
  note: OUTPUTS AND MONITORING
  demand : Inport  PortDimensions=3
  parameters : Inport  Port=2  PortDimensions=52
  Hydrogen chemical energy consumed kWh : Fcn  Expr=u(1)*u(2)
  Hydrogen used each second kg : Fcn  Expr=u(1)/(3600*(((u(2))+(0.000001)+abs((u(2))-(0.000001)))/2))
  Usable hydrogen remaining kg : Fcn  Expr=((u(1)-u(2))+abs(u(1)-u(2)))/2
  chemical : Fcn  Expr=u(2)
  combine Inventory : Mux  Inputs=3
  h2_initial : Fcn  Expr=u(35)
  h2_lhv : Fcn  Expr=u(36)
  inputs energy : Mux  Inputs=2
  inputs remaining : Mux  Inputs=2
  inputs step_mass : Mux  Inputs=2
  inputs used_next : Mux  Inputs=2
  used : UnitDelay
  used accumulation : Fcn  Expr=u(1)+u(2)
  Inventory : Outport  PortDimensions=3
  wires:
  [parameters] -> h2_lhv/1
  Hydrogen chemical energy consumed kWh/1 -> [energy]
  [used] -> combine Inventory/2
  [demand] -> chemical/1
  [used] -> inputs energy/1
  [remaining] -> combine Inventory/1
  [parameters] -> h2_initial/1
  [energy] -> combine Inventory/3
  parameters/1 -> [parameters]
  [h2_lhv] -> inputs energy/2
  [used_next] -> used/1
  demand/1 -> [demand]
  [chemical] -> inputs step_mass/1
  [h2_lhv] -> inputs step_mass/2
  [used] -> inputs used_next/1
  [step_mass] -> inputs used_next/2
  [h2_initial] -> inputs remaining/1
  [used] -> inputs remaining/2
  h2_lhv/1 -> [h2_lhv]
  chemical/1 -> [chemical]
  combine Inventory/1 -> Inventory/1
  used accumulation/1 -> [used_next]
  h2_initial/1 -> [h2_initial]
  inputs energy/1 -> Hydrogen chemical energy consumed kWh/1
  used/1 -> [used]
  inputs step_mass/1 -> Hydrogen used each second kg/1
  inputs used_next/1 -> used accumulation/1
  inputs remaining/1 -> Usable hydrogen remaining kg/1
  Hydrogen used each second kg/1 -> [step_mass]
  Usable hydrogen remaining kg/1 -> [remaining]

== system Powertrain_Comparison/Electric powertrain/Inverter ==
  note: Inverter
  note: INVERTER | average power conversion
      | DC to AC in motoring; AC to DC during regeneration. Efficiency is an editable assumption; switching waveforms are excluded.
  note: INPUT SIGNALS
  note: PARAMETERS AND SIGNAL SELECTION
  note: CALCULATIONS AND CONTROL
  note: OUTPUTS AND MONITORING
  demand : Inport  PortDimensions=9
  parameters : Inport  Port=2  PortDimensions=52
  DC demand kW positive motoring : Fcn  Expr=(u(1)>=0)*u(1)/(((u(2))+(0.000001)+abs((u(2))-(0.000001)))/2)+(u(1)<0)*u(1)*u(2)
  Inverter conversion loss kW : Fcn  Expr=((u(1)-u(2))+abs(u(1)-u(2)))/2
  Unused diagnostic shaft : Terminator
  ac : Fcn  Expr=u(1)
  combine Inverter signals : Mux  Inputs=2
  eta_inv : Fcn  Expr=u(26)
  inputs dc : Mux  Inputs=2
  inputs loss : Mux  Inputs=2
  shaft : Fcn  Expr=u(2)
  Inverter signals : Outport  PortDimensions=2
  wires:
  demand/1 -> [demand]
  [demand] -> shaft/1
  [parameters] -> eta_inv/1
  [demand] -> ac/1
  DC demand kW positive motoring/1 -> [dc]
  [ac] -> inputs dc/1
  [dc] -> inputs loss/1
  parameters/1 -> [parameters]
  [eta_inv] -> inputs dc/2
  [ac] -> inputs loss/2
  [dc] -> combine Inverter signals/1
  [loss] -> combine Inverter signals/2
  shaft/1 -> Unused diagnostic shaft/1
  ac/1 -> [ac]
  eta_inv/1 -> [eta_inv]
  inputs dc/1 -> DC demand kW positive motoring/1
  inputs loss/1 -> Inverter conversion loss kW/1
  combine Inverter signals/1 -> Inverter signals/1
  Inverter conversion loss kW/1 -> [loss]

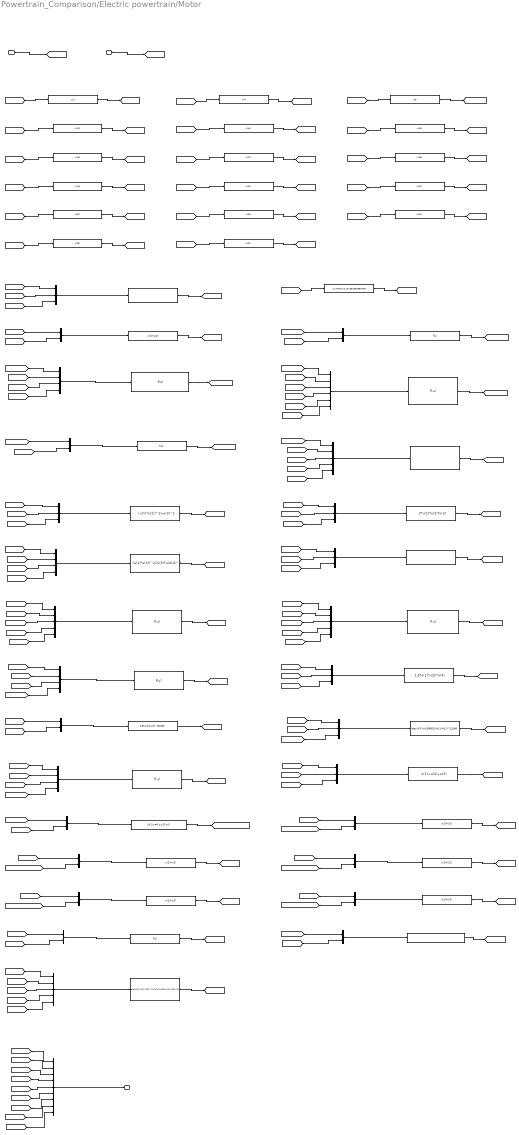
== system Powertrain_Comparison/Electric powertrain/Motor ==
  note: Motor
  note: ELECTRIC MOTOR | steady-state adaptation of the saved PMSM model
      | Reused: Te = 1.5 p psi iq, vd = -omega_e Lq iq, vq = Rs iq + omega_e psi, copper loss = 1.5 Rs iq^2.
      | Current-area scaling 7.8125: Imax 80 to 625 A; Rs and L divided by 7.8125. Assumed 120 kW-class design, not a calibrated
      | motor.
  note: INPUT SIGNALS
  note: PARAMETERS AND SIGNAL SELECTION
  note: CALCULATIONS AND CONTROL
  note: OUTPUTS AND MONITORING
  demand : Inport  PortDimensions=9
  parameters : Inport  Port=2  PortDimensions=52
  Active ac : Fcn  Expr=u(1)*u(2)
  Active copper : Fcn  Expr=u(1)*u(2)
  Active iq : Fcn  Expr=u(1)*u(2)
  Active shaft : Fcn  Expr=u(1)*u(2)
  Active viscous : Fcn  Expr=u(1)*u(2)
  Available generating iq magnitude A : Fcn  Expr=(u(4)<=0)*(((u(5))+((((u(2)+u(3))/(2*(((u(1))+(0.000001)+abs((u(1))-(0.000001)))/2)))+abs((u(2)+u(3))/(2*(((u(1))+(0.000001)+abs((u(1))-(0.000001)))/2))))/2)-abs((u(5))-((((u(2)+u(3))/(2*(((u(1))+(0.000001)+abs((u(1))-(0.000001)))/2)))+abs((u(2)+u(3))/(2*(((u(1))+(0.000001)+abs((u(1))-(0.000001)))/2))))/2)))/2)
  Available motoring iq A : Fcn  Expr=(u(4)<=0)*(((u(5))+((((-u(2)+u(3))/(2*(((u(1))+(0.000001)+abs((u(1))-(0.000001)))/2)))+abs((-u(2)+u(3))/(2*(((u(1))+(0.000001)+abs((u(1))-(0.000001)))/2))))/2)-abs((u(5))-((((-u(2)+u(3))/(2*(((u(1))+(0.000001)+abs((u(1))-(0.000001)))/2)))+abs((-u(2)+u(3))/(2*(((u(1))+(0.000001)+abs((u(1))-(0.000001)))/2))))/2)))/2)
  Available shaft power kW : Fcn  Expr=(u(4)>=0)*(((u(1)*u(2)/1000-u(3))+abs(u(1)*u(2)/1000-u(3)))/2)+(u(4)<0)*(u(1)*u(2)/1000-u(3))
  Copper loss kW : Fcn  Expr=1.5*u(1)*u(2)^2/1000
  Electrical angular speed rad per s : Fcn  Expr=u(1)*u(2)
  Electromagnetic torque Nm : Fcn  Expr=1.5*u(1)*u(2)*u(3)
  Limited motor iq A : Fcn  Expr=(abs(u(4))>0.000001)*(((((u(1))+(-u(3))+abs((u(1))-(-u(3))))/2)+(u(2))-abs((((u(1))+(-u(3))+abs((u(1))-(-u(3))))/2)-(u(2))))/2)
  Mechanical angular speed rad per s : Fcn  Expr=u(1)*u(2)/(((u(3))+(0.000001)+abs((u(3))-(0.000001)))/2)
  Motor AC active power kW : Fcn  Expr=u(1)+u(2)+u(3)
  Motor speed rpm : Fcn  Expr=u(1)*60/(2*3.141592653589793)
  Motor-limited wheel power kW : Fcn  Expr=(u(1)>=0)*u(1)*u(2)+(u(1)<0)*u(1)/(((u(2))+(0.000001)+abs((u(2))-(0.000001)))/2)
  Motoring or net regenerative operation : Fcn  Expr=(u(1)>=0 || u(2)<0)
  PMSM requested iq A with id zero : Fcn  Expr=(u(1)+u(2)*u(3))/(1.5*(((u(4)*u(5))+(0.000001)+abs((u(4)*u(5))-(0.000001)))/2))
  Peak power and regenerative power limits : Fcn  Expr=((((u(1))+(-u(3)*u(4))+abs((u(1))-(-u(3)*u(4))))/2)+(u(2))-abs((((u(1))+(-u(3)*u(4))+abs((u(1))-(-u(3)*u(4))))/2)-(u(2))))/2
  Peak shaft torque limit Nm : Fcn  Expr=((((u(1))+(-u(2))+abs((u(1))-(-u(2))))/2)+(u(2))-abs((((u(1))+(-u(2))+abs((u(1))-(-u(2))))/2)-(u(2))))/2
  Requested shaft power kW : Fcn  Expr=(u(1)>=0)*u(1)/(((u(2))+(0.000001)+abs((u(2))-(0.000001)))/2)+(u(1)<0)*u(1)*u(2)
  Required dq voltage magnitude V : Fcn  Expr=sqrt((u(1)*u(2)*u(3))^2+(u(4)*u(3)+u(1)*u(5))^2)
  Required shaft torque Nm : Fcn  Expr=(u(2)>0.0001)*u(1)*1000/(((u(2))+(0.000001)+abs((u(2))-(0.000001)))/2)+(u(2)<=0.0001)*u(3)*u(4)/((((u(5)*u(6))+(0.000001)+abs((u(5)*u(6))-(0.000001)))/2))
  Viscous loss kW : Fcn  Expr=(abs(u(3))>0.000001)*u(1)*u(2)^2/1000
  Voltage constraint coefficient A : Fcn  Expr=(u(1)*u(2))^2+u(3)^2
  Voltage constraint coefficient B : Fcn  Expr=2*u(1)*u(2)*u(3)
  Voltage constraint coefficient C : Fcn  Expr=(u(1)*u(2))^2-(u(3)*u(4)/2)^2
  Voltage limit discriminant : Fcn  Expr=sqrt(((u(2)^2-4*u(1)*u(3))+abs(u(2)^2-4*u(1)*u(3)))/2)
  Wheel demand beyond motor capability kW : Fcn  Expr=((((u(1))+abs(u(1)))/2-((u(2))+abs(u(2)))/2)+abs(((u(1))+abs(u(1)))/2-((u(2))+abs(u(2)))/2))/2
  b : Fcn  Expr=u(22)
  combine Motor signals : Mux  Inputs=9
  eta_gear : Fcn  Expr=u(15)
  flux : Fcn  Expr=u(19)
  force : Fcn  Expr=u(4)
  gear : Fcn  Expr=u(14)
  imax : Fcn  Expr=u(23)
  inputs a_voltage : Mux  Inputs=3
  inputs ac : Mux  Inputs=2
  inputs ac_raw : Mux  Inputs=3
  inputs b_voltage : Mux  Inputs=3
  inputs c_voltage : Mux
  inputs copper : Mux  Inputs=2
  inputs copper_raw : Mux  Inputs=2
  inputs electrical_brake_enabled : Mux  Inputs=2
  inputs iq : Mux  Inputs=2
  inputs iq_neg : Mux  Inputs=5
  inputs iq_pos : Mux  Inputs=5
  inputs iq_raw : Mux
  inputs iq_request : Mux  Inputs=5
  inputs omega : Mux  Inputs=3
  inputs omega_e : Mux  Inputs=2
  inputs phase_v : Mux  Inputs=5
  inputs root_voltage : Mux  Inputs=3
  inputs shaft : Mux  Inputs=2
  inputs shaft_limited : Mux
  inputs shaft_raw : Mux
  inputs shaft_request : Mux  Inputs=2
  inputs te : Mux  Inputs=3
  inputs torque_limited : Mux  Inputs=2
  inputs torque_request : Mux  Inputs=6
  inputs unmet_motor : Mux  Inputs=2
  inputs viscous : Mux  Inputs=2
  inputs viscous_raw : Mux  Inputs=3
  inputs wheel_cap : Mux  Inputs=2
  lq : Fcn  Expr=u(21)
  mod : Fcn  Expr=u(24)
  motor_kw : Fcn  Expr=u(16)
  pole : Fcn  Expr=u(18)
  radius : Fcn  Expr=u(13)
  regen_kw : Fcn  Expr=u(37)
  rs : Fcn  Expr=u(20)
  torque : Fcn  Expr=u(17)
  v : Fcn  Expr=u(1)
  vbus : Fcn  Expr=u(25)
  wheel_request : Fcn  Expr=u(5)
  Motor signals : Outport  PortDimensions=9
  wires:
  [shaft] -> inputs wheel_cap/1
  Active shaft/1 -> [shaft]
  [viscous_raw] -> inputs shaft_raw/3
  [parameters] -> vbus/1
  [copper] -> combine Motor signals/3
  inputs iq_request/1 -> PMSM requested iq A with id zero/1
  eta_gear/1 -> [eta_gear]
  [viscous_raw] -> inputs viscous/1
  [phase_v] -> combine Motor signals/7
  combine Motor signals/1 -> Motor signals/1
  parameters/1 -> [parameters]
  [shaft_limited] -> inputs torque_request/1
  Available motoring iq A/1 -> [iq_pos]
  [wheel_cap] -> combine Motor signals/9
  [iq] -> combine Motor signals/6
  [flux] -> inputs b_voltage/3
  [viscous] -> combine Motor signals/4
  [rpm] -> combine Motor signals/5
  [shaft_raw] -> inputs ac_raw/1
  inputs ac_raw/1 -> Motor AC active power kW/1
  inputs copper/1 -> Active copper/1
  inputs shaft/1 -> Active shaft/1
  [unmet_motor] -> combine Motor signals/8
  [parameters] -> eta_gear/1
  inputs shaft_raw/1 -> Available shaft power kW/1
  [shaft] -> combine Motor signals/2
  [copper_raw] -> inputs ac_raw/2
  [ac] -> combine Motor signals/1
  Required dq voltage magnitude V/1 -> [phase_v]
  [wheel_cap] -> inputs unmet_motor/2
  inputs phase_v/1 -> Required dq voltage magnitude V/1
  [flux] -> inputs phase_v/5
  [omega] -> inputs shaft_raw/2
  [rs] -> inputs phase_v/4
  [iq] -> inputs phase_v/3
  [force] -> inputs torque_request/3
  [parameters] -> torque/1
  [electrical_brake_enabled] -> inputs copper/2
  mod/1 -> [mod]
  [lq] -> inputs phase_v/2
  Active copper/1 -> [copper]
  [omega_e] -> inputs phase_v/1
  inputs iq/1 -> Active iq/1
  Wheel demand beyond motor capability kW/1 -> [unmet_motor]
  [demand] -> force/1
  inputs unmet_motor/1 -> Wheel demand beyond motor capability kW/1
  [omega] -> inputs torque_request/2
  [wheel_request] -> inputs unmet_motor/1
  Motor-limited wheel power kW/1 -> [wheel_cap]
  inputs ac/1 -> Active ac/1
  lq/1 -> [lq]
  [shaft_raw] -> inputs shaft/1
  [parameters] -> gear/1
  inputs wheel_cap/1 -> Motor-limited wheel power kW/1
  [iq_raw] -> inputs iq/1
  [a_voltage] -> inputs root_voltage/1
  [eta_gear] -> inputs wheel_cap/2
  [copper_raw] -> inputs copper/1
  Active ac/1 -> [ac]
  [electrical_brake_enabled] -> inputs ac/2
  Active viscous/1 -> [viscous]
  [electrical_brake_enabled] -> inputs viscous/2
  [ac_raw] -> inputs ac/1
  [electrical_brake_enabled] -> inputs shaft/2
  [electrical_brake_enabled] -> inputs iq/2
  inputs viscous/1 -> Active viscous/1
  Active iq/1 -> [iq]
  Motoring or net regenerative operation/1 -> [electrical_brake_enabled]
  inputs electrical_brake_enabled/1 -> Motoring or net regenerative operation/1
  inputs a_voltage/1 -> Voltage constraint coefficient A/1
  [ac_raw] -> inputs electrical_brake_enabled/2
  [flux] -> inputs c_voltage/2
  [shaft_request] -> inputs electrical_brake_enabled/1
  [rs] -> inputs a_voltage/3
  Motor AC active power kW/1 -> [ac_raw]
  [te] -> inputs shaft_raw/1
  [viscous_raw] -> inputs ac_raw/3
  Available shaft power kW/1 -> [shaft_raw]
  [shaft_limited] -> inputs shaft_raw/4
  inputs copper_raw/1 -> Copper loss kW/1
  Viscous loss kW/1 -> [viscous_raw]
  inputs viscous_raw/1 -> Viscous loss kW/1
  gear/1 -> [gear]
  [wheel_request] -> inputs viscous_raw/3
  [omega] -> inputs viscous_raw/2
  [b] -> inputs viscous_raw/1
  [radius] -> inputs torque_request/4
  Copper loss kW/1 -> [copper_raw]
  rs/1 -> [rs]
  [iq_raw] -> inputs copper_raw/2
  [rs] -> inputs copper_raw/1
  Electromagnetic torque Nm/1 -> [te]
  inputs te/1 -> Electromagnetic torque Nm/1
  [iq_raw] -> inputs te/3
  [flux] -> inputs te/2
  [pole] -> inputs te/1
  Limited motor iq A/1 -> [iq_raw]
  PMSM requested iq A with id zero/1 -> [iq_request]
  inputs iq_raw/1 -> Limited motor iq A/1
  [wheel_request] -> inputs iq_raw/4
  [iq_neg] -> inputs iq_raw/3
  [iq_pos] -> inputs iq_raw/2
  [iq_request] -> inputs iq_raw/1
  Available generating iq magnitude A/1 -> [iq_neg]
  [c_voltage] -> inputs root_voltage/3
  inputs iq_neg/1 -> Available generating iq magnitude A/1
  [imax] -> inputs iq_neg/5
  [c_voltage] -> inputs iq_neg/4
  [root_voltage] -> inputs iq_neg/3
  [b_voltage] -> inputs iq_neg/2
  [a_voltage] -> inputs iq_neg/1
  inputs iq_pos/1 -> Available motoring iq A/1
  [imax] -> inputs iq_pos/5
  [b_voltage] -> inputs iq_pos/2
  [c_voltage] -> inputs iq_pos/4
  [root_voltage] -> inputs iq_pos/3
  [a_voltage] -> inputs iq_pos/1
  inputs shaft_request/1 -> Requested shaft power kW/1
  Voltage limit discriminant/1 -> [root_voltage]
  [eta_gear] -> inputs torque_request/6
  inputs root_voltage/1 -> Voltage limit discriminant/1
  [parameters] -> motor_kw/1
  inputs b_voltage/1 -> Voltage constraint coefficient B/1
  [b_voltage] -> inputs root_voltage/2
  Voltage constraint coefficient C/1 -> [c_voltage]
  imax/1 -> [imax]
  inputs c_voltage/1 -> Voltage constraint coefficient C/1
  [vbus] -> inputs c_voltage/4
  [mod] -> inputs c_voltage/3
  pole/1 -> [pole]
  [omega_e] -> inputs c_voltage/1
  Voltage constraint coefficient B/1 -> [b_voltage]
  [omega_e] -> inputs b_voltage/2
  [rs] -> inputs b_voltage/1
  Voltage constraint coefficient A/1 -> [a_voltage]
  [lq] -> inputs a_voltage/2
  [omega_e] -> inputs a_voltage/1
  b/1 -> [b]
  [flux] -> inputs iq_request/5
  [pole] -> inputs iq_request/4
  [omega] -> inputs iq_request/3
  [b] -> inputs iq_request/2
  [torque_limited] -> inputs iq_request/1
  Peak shaft torque limit Nm/1 -> [torque_limited]
  inputs torque_limited/1 -> Peak shaft torque limit Nm/1
  [torque] -> inputs torque_limited/2
  [torque_request] -> inputs torque_limited/1
  Required shaft torque Nm/1 -> [torque_request]
  vbus/1 -> [vbus]
  inputs torque_request/1 -> Required shaft torque Nm/1
  [gear] -> inputs torque_request/5
  Peak power and regenerative power limits/1 -> [shaft_limited]
  [eta_gear] -> inputs shaft_request/2
  inputs shaft_limited/1 -> Peak power and regenerative power limits/1
  [eta_gear] -> inputs shaft_limited/4
  [regen_kw] -> inputs shaft_limited/3
  [motor_kw] -> inputs shaft_limited/2
  [shaft_request] -> inputs shaft_limited/1
  Requested shaft power kW/1 -> [shaft_request]
  [wheel_request] -> inputs shaft_request/1
  Electrical angular speed rad per s/1 -> [omega_e]
  inputs omega_e/1 -> Electrical angular speed rad per s/1
  [pole] -> inputs omega_e/2
  [omega] -> inputs omega_e/1
  Motor speed rpm/1 -> [rpm]
  [omega] -> Motor speed rpm/1
  Mechanical angular speed rad per s/1 -> [omega]
  inputs omega/1 -> Mechanical angular speed rad per s/1
  [radius] -> inputs omega/3
  [gear] -> inputs omega/2
  torque/1 -> [torque]
  [v] -> inputs omega/1
  regen_kw/1 -> [regen_kw]
  [parameters] -> regen_kw/1
  [parameters] -> mod/1
  [parameters] -> imax/1
  [parameters] -> b/1
  [parameters] -> lq/1
  [parameters] -> rs/1
  flux/1 -> [flux]
  [parameters] -> flux/1
  [parameters] -> pole/1
  motor_kw/1 -> [motor_kw]
  radius/1 -> [radius]
  [parameters] -> radius/1
  wheel_request/1 -> [wheel_request]
  [demand] -> wheel_request/1
  force/1 -> [force]
  v/1 -> [v]
  [demand] -> v/1
  demand/1 -> [demand]
